simulink model "Robot_2R_Dynamics_and_Control"  (R2025a)
settings: Solver=ode4  StartTime=0.0  StopTime=stpt  FixedStep=0.001  MaxStep=0.001  MinStep=1e-6  RelTol=1e-3
undefined symbols (not defined in the file): acceleration, c, position, velocity, x, xx
libraries: slpidlib x2
settings Model: SimulationMode=accelerator  Creator=davi_  LastModifiedBy=GrupoGarra
settings DebuggingCC: UnconnectedInputMsg=warning  UnconnectedOutputMsg=warning  UnconnectedLineMsg=warning
settings ModelReferenceCC: EnableRefExpFcnMdlSchedulingChecks=on
settings RTWCC: GPUComputeCapability=3.5  DLArmComputeVersion=19.05

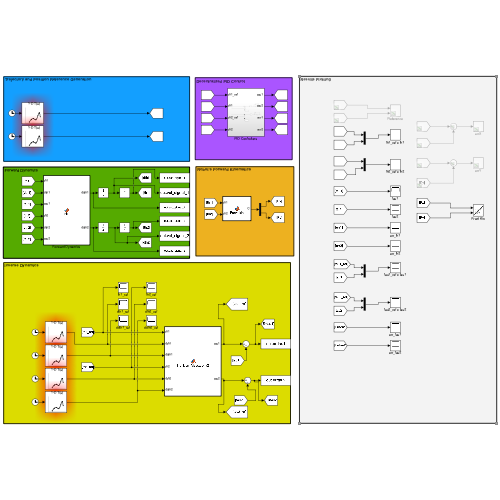
[thumbnail: Simulink's stored preview of the top-level diagram]
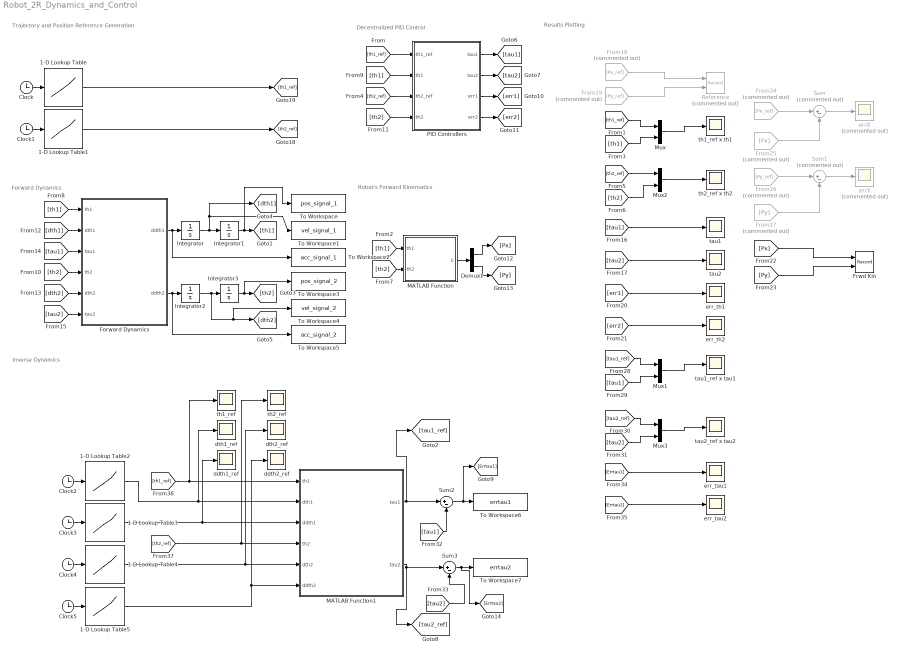
== system Robot_2R_Dynamics_and_Control ==
  note: Inverse Dynamics
  note: Results Plotting
  note: Forward Dynamics
  note: Robot's Forward Kinematics
  note: Trajectory and Position Reference Generation
  note: Decentralized PID Control
  1-D Lookup Table : Lookup_n-D  NumberOfTableDimensions=1  BreakpointsForDimension1=xx  Table=position(1,:)  InterpMethod=Cubic spline  ExtrapMethod=Clip  InternalRulePriority=Speed  RndMeth=Simplest
  1-D Lookup Table1 : Lookup_n-D  NumberOfTableDimensions=1  BreakpointsForDimension1=xx  Table=position(2,:)  InterpMethod=Cubic spline  ExtrapMethod=Clip  InternalRulePriority=Speed  RndMeth=Simplest
  1-D Lookup Table2 : Lookup_n-D  NumberOfTableDimensions=1  BreakpointsForDimension1=xx  Table=velocity(1,:)  InterpMethod=Cubic spline  ExtrapMethod=Clip  InternalRulePriority=Speed  RndMeth=Simplest
  1-D Lookup Table3 : Lookup_n-D  NumberOfTableDimensions=1  BreakpointsForDimension1=xx  Table=acceleration(1,:)  InterpMethod=Cubic spline  ExtrapMethod=Clip  InternalRulePriority=Speed  RndMeth=Simplest
  1-D Lookup Table4 : Lookup_n-D  NumberOfTableDimensions=1  BreakpointsForDimension1=xx  Table=velocity(2,:)  InterpMethod=Cubic spline  ExtrapMethod=Clip  InternalRulePriority=Speed  RndMeth=Simplest
  1-D Lookup Table5 : Lookup_n-D  NumberOfTableDimensions=1  BreakpointsForDimension1=xx  Table=acceleration(2,:)  InterpMethod=Cubic spline  ExtrapMethod=Clip  InternalRulePriority=Speed  RndMeth=Simplest
  Clock{,1..5} (6 alike) : Clock
  Demux1 : Demux  Outputs=2
  Forward Dynamics : MATLAB Function  TreatAsAtomicUnit=on
  From18 : From  Commented=on  GotoTag=Px_ref
  From19 : From  Commented=on  GotoTag=Py_ref
  From24 : From  Commented=on  GotoTag=Px_ref
  From25 : From  Commented=on  GotoTag=Px
  From26 : From  Commented=on  GotoTag=Py_ref
  From27 : From  Commented=on  GotoTag=Py
  Frwd Kin : Record  NumPorts=2.0  FileSettingsInternal="{\"entries\":[{\"content\":{\"excelSettings\":{\"content\":{},\"type\":\"Streamout.ExcelSettings\"},\"parquetSettings\":{\"content\":{},\"type\":\"Streamout.ParquetSettings\"}},\"type\":\"Streamout.FileSettingStorage\",\"uuid\":\"\"}],\"packageUris\":[\"http:\\/\\/schema.mathworks.com\\/mf0\\/streamout_blocks\\/R2020a\"],\"version\":\"1.0\"}"  FrameSettings=[0, 0]  Layout=[1 1]  SignalsInternal="{\"entries\":[{\"content\":{\"signals\":[{\"content\":{\"blockPath\":[],\"dimensions\":[1],\"domain\":\"\",\"lineColor\":\"#a2142f\",\"plots\":[ 1 ],\"port\":1,\"signalID\":1,\"signalName\":\"From22\"},\"type\":\"RecordBlkView.Signal\",\"uuid\":\"\"},{\"content\":{\"blockPath\":[],\"dimensions\":[1],\"domain\":\"\",\"lineColor\":\"#139fff\",\"plots\":[ 1 ],\"port\":2,\"signalID\":2,\"signalName\":\"From23\"},\"type\":\"RecordBlkView.Signal\",\"uuid\":\"\"}]},\"type\":\"RecordBlkView.InputSignals\",\"uuid\":\"\"}],\"packageUris\":[\"http:\\/\\/schema.mathworks.com\\/mf0\\/streamout_blocks\\/R2020a\"],\"version\":\"1.0\"}"  VisualizationBindings="{\"xyplotplugin\":{\"info\":[{\"series\":[{\"bindingParametersList\":[{\"parameter\":\"X-Axis\",\"signalID\":1,\"signalName\":\"From22\"},{\"parameter\":\"Y-Axis\",\"signalID\":2,\"signalName\":\"From23\"}],\"seriesID\":0}],\"subplotID\":1}]}}"  CompatibilityTag=XY  st=-1
  Integrator{,1..3} (4 alike) : Integrator
  MATLAB Function : MATLAB Function  TreatAsAtomicUnit=on
  MATLAB Function1 : MATLAB Function  TreatAsAtomicUnit=on
  Mux{,1..3} (4 alike) : Mux  Inputs=2
  PID Controllers : Subsystem
  Reference : Record  Commented=on  NumPorts=2.0  FileSettingsInternal="{\"entries\":[{\"content\":{\"excelSettings\":{\"content\":{},\"type\":\"Streamout.ExcelSettings\"},\"parquetSettings\":{\"content\":{},\"type\":\"Streamout.ParquetSettings\"}},\"type\":\"Streamout.FileSettingStorage\",\"uuid\":\"\"}],\"packageUris\":[\"http:\\/\\/schema.mathworks.com\\/mf0\\/streamout_blocks\\/R2020a\"],\"version\":\"1.0\"}"  FrameSettings=[0, 0]  Layout=[1 1]  SignalsInternal="{\"entries\":[{\"content\":{\"signals\":[{\"content\":{\"blockPath\":[],\"dimensions\":[1],\"domain\":\"\",\"lineColor\":\"#a2142f\",\"plots\":[ 1 ],\"port\":1,\"signalID\":1,\"signalName\":\"XY Graph:1\"},\"type\":\"RecordBlkView.Signal\",\"uuid\":\"\"},{\"content\":{\"blockPath\":[],\"dimensions\":[1],\"domain\":\"\",\"lineColor\":\"#139fff\",\"plots\":[ 1 ],\"port\":2,\"signalID\":2,\"signalName\":\"XY Graph:2\"},\"type\":\"RecordBlkView.Signal\",\"uuid\":\"\"}]},\"type\":\"RecordBlkView.InputSignals\",\"uuid\":\"\"}],\"packageUris\":[\"http:\\/\\/schema.mathworks.com\\/mf0\\/streamout_blocks\\/R2020a\"],\"version\":\"1.0\"}"  VisualizationBindings="{\"xyplotplugin\":{\"info\":[{\"series\":[{\"bindingParametersList\":[{\"parameter\":\"X-Axis\",\"signalID\":1,\"signalName\":\"XY Graph:1\"},{\"parameter\":\"Y-Axis\",\"signalID\":2,\"signalName\":\"XY Graph:2\"}],\"seriesID\":0}],\"subplotID\":1}]}}"  CompatibilityTag=XY  st=-1
  Sum : Sum  Commented=on  Inputs=|+-
  Sum1 : Sum  Commented=on  Inputs=|+-
  Sum2 : Sum  Inputs=|+-
  Sum3 : Sum  Inputs=|+-
  To Workspace : ToWorkspace  VariableName=pos_signal_1  SampleTime=-1
  To Workspace1 : ToWorkspace  VariableName=vel_signal_1  SampleTime=-1
  To Workspace2 : ToWorkspace  VariableName=acc_signal_1  SampleTime=-1
  To Workspace3 : ToWorkspace  VariableName=pos_signal_2  SampleTime=-1
  To Workspace4 : ToWorkspace  VariableName=vel_signal_2  SampleTime=-1
  To Workspace5 : ToWorkspace  VariableName=acc_signal_2  SampleTime=-1
  To Workspace6 : ToWorkspace  VariableName=errtau1  SampleTime=-1
  To Workspace7 : ToWorkspace  VariableName=errtau2  SampleTime=-1
  ddth1_ref : Scope
      settings: ActiveDisplayYMinimum=-1.7046  ActiveDisplayYMaximum=10.72886  DataLoggingVariableName=ScopeData2
  ddth2_ref : Scope
      settings: ActiveDisplayYMinimum=-29.79825  ActiveDisplayYMaximum=6.00469  DataLoggingVariableName=ScopeData3
  dth1_ref : Scope
      settings: ActiveDisplayYMinimum=-0.76549  ActiveDisplayYMaximum=1.78872
  dth2_ref : Scope
      settings: ActiveDisplayYMinimum=-0.46079  ActiveDisplayYMaximum=1.47482  DataLoggingVariableName=ScopeData5
  errX : Scope  Commented=on
      settings: ActiveDisplayYMinimum=-0.05671  ActiveDisplayYMaximum=0.09104  DataLoggingVariableName=ScopeData5
  errY : Scope  Commented=on
      settings: ActiveDisplayYMinimum=-0.05671  ActiveDisplayYMaximum=0.09104  DataLoggingVariableName=ScopeData6
  err_tau1 : Scope
      settings: ActiveDisplayYMinimum=-0.10365664078186178  ActiveDisplayYMaximum=0.12157927180851377
  err_tau2 : Scope
      settings: ActiveDisplayYMinimum=-0.11596  ActiveDisplayYMaximum=0.12339  DataLoggingVariableName=ScopeData2
  err_th1 : Scope
      settings: ActiveDisplayYMinimum=-0.0011718016150849826  ActiveDisplayYMaximum=0.000974877138754193  DataLoggingVariableName=ScopeData2
  err_th2 : Scope
      settings: ActiveDisplayYMinimum=-0.46542  ActiveDisplayYMaximum=0.0529
  tau1 : Scope
      settings: ActiveDisplayYMinimum=-21.92284  ActiveDisplayYMaximum=23.22624  DataLoggingVariableName=ScopeData3
  tau1_ref x tau1 : Scope
      settings: ActiveDisplayYMinimum=-22.72078  ActiveDisplayYMaximum=23.87515
  tau2 : Scope
      settings: ActiveDisplayYMinimum=-3.67368  ActiveDisplayYMaximum=4.67521  DataLoggingVariableName=ScopeData4
  tau2_ref x tau2 : Scope
      settings: ActiveDisplayYMinimum=-16.2578  ActiveDisplayYMaximum=18.66466  DataLoggingVariableName=ScopeData2
  th1_ref : Scope
      settings: ActiveDisplayYMinimum=-0.4737  ActiveDisplayYMaximum=1.16382  DataLoggingVariableName=ScopeData3
  th1_ref x th1 : Scope
      settings: ActiveDisplayYMinimum=-0.47526  ActiveDisplayYMaximum=1.16405
  th2_ref : Scope
      settings: ActiveDisplayYMinimum=-0.98175  ActiveDisplayYMaximum=0.98175  DataLoggingVariableName=ScopeData4
  th2_ref x th2 : Scope
      settings: ActiveDisplayYMinimum=-0.14358  ActiveDisplayYMaximum=1.2922  DataLoggingVariableName=ScopeData7
  wires:
  Forward Dynamics/1(ddth1) -> To Workspace2/1, Integrator/1
  Integrator/1 -> To Workspace1/1, [dth1], Integrator1/1
  Integrator1/1 -> To Workspace/1, [th1]
  Forward Dynamics/2(ddth2) -> To Workspace5/1, Integrator2/1
  Integrator2/1 -> To Workspace4/1, [dth2], Integrator3/1
  Integrator3/1 -> To Workspace3/1, [th2]
  Mux/1 -> th1_ref x th1/1
  Sum/1 -> errX/1
  Sum1/1 -> errY/1
  [th1_ref] -> Mux/1
  [th1] -> MATLAB Function/1(th1)
  [th1] -> Mux/2
  [th2] -> Mux2/2
  [th2_ref] -> Mux2/1
  Mux2/1 -> th2_ref x th2/1
  [th2] -> MATLAB Function/2(th2)
  [th1] -> Forward Dynamics/1(th1)
  [th2] -> Forward Dynamics/4(th2)
  [dth1] -> Forward Dynamics/2(dth1)
  [dth2] -> Forward Dynamics/5(dth2)
  [tau1] -> Forward Dynamics/3(tau1)
  [tau2] -> Forward Dynamics/6(tau2)
  [tau1] -> tau1/1
  [tau2] -> tau2/1
  From18/1 -> Reference/1
  From19/1 -> Reference/2
  [err1] -> err_th1/1
  [err2] -> err_th2/1
  MATLAB Function/1(C) -> Demux1/1
  Demux1/2 -> [Py]
  Demux1/1 -> [Px]
  [Px] -> Frwd Kin/1
  [Py] -> Frwd Kin/2
  From24/1 -> Sum/1
  From25/1 -> Sum/2
  From26/1 -> Sum1/1
  From27/1 -> Sum1/2
  PID Controllers/4(err2) -> [err2]
  [th2] -> PID Controllers/4(th2)
  PID Controllers/1(tau1) -> [tau1]
  PID Controllers/2(tau2) -> [tau2]
  [th1_ref] -> PID Controllers/1(th1_ref)
  PID Controllers/3(err1) -> [err1]
  [th2_ref] -> PID Controllers/3(th2_ref)
  [th1] -> PID Controllers/2(th1)
  1-D Lookup Table/1 -> [th1_ref]
  1-D Lookup Table1/1 -> [th2_ref]
  1-D Lookup Table2/1 -> MATLAB Function1/2(dth1), dth1_ref/1
  MATLAB Function1/2(tau2) -> Sum3/1, [tau2_ref]
  1-D Lookup Table4/1 -> MATLAB Function1/5(dth2), dth2_ref/1
  [th2_ref] -> th2_ref/1, MATLAB Function1/4(th2)
  1-D Lookup Table5/1 -> MATLAB Function1/6(ddth2), ddth2_ref/1
  1-D Lookup Table3/1 -> MATLAB Function1/3(ddth1), ddth1_ref/1
  MATLAB Function1/1(tau1) -> Sum2/1, [tau1_ref]
  [tau1_ref] -> Mux1/1
  [tau1] -> Mux1/2
  Mux1/1 -> tau1_ref x tau1/1
  Mux3/1 -> tau2_ref x tau2/1
  [tau2] -> Mux3/2
  [tau2_ref] -> Mux3/1
  [tau1] -> Sum2/2
  [tau2] -> Sum3/2
  Sum2/1 -> To Workspace6/1, [Errtau1]
  Sum3/1 -> To Workspace7/1, [Errtau2]
  [Errtau2] -> err_tau2/1
  [Errtau1] -> err_tau1/1
  Clock/1 -> 1-D Lookup Table/1
  Clock1/1 -> 1-D Lookup Table1/1
  [th1_ref] -> th1_ref/1, MATLAB Function1/1(th1)
  Clock2/1 -> 1-D Lookup Table2/1
  Clock3/1 -> 1-D Lookup Table3/1
  Clock4/1 -> 1-D Lookup Table4/1
  Clock5/1 -> 1-D Lookup Table5/1

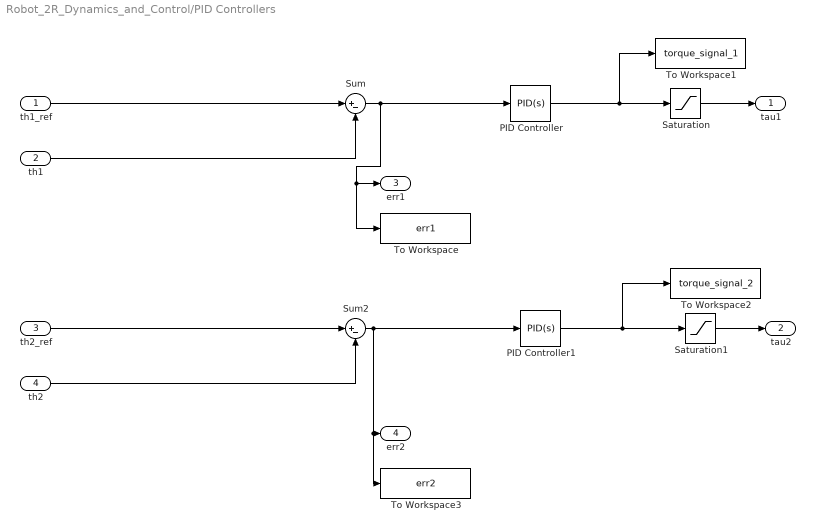
== system Robot_2R_Dynamics_and_Control/PID Controllers ==
  th1_ref : Inport
  th1 : Inport  Port=2
  th2_ref : Inport  Port=3
  th2 : Inport  Port=4
  PID Controller : slpidlib/PID Controller  Controller=PID  Form=Parallel  TimeDomain=Continuous-time  UseExternalTs=off  SampleTime=-1  IntegratorMethod=Forward Euler  FilterMethod=Forward Euler  ControllerParametersSource=internal  P=x(1)  I=x(3)  UseKiTs=off  D=x(2)  UseExternalDerivativeSource=off  N=c  UseFilter=on  TunerSelectOption=Transfer Function Based (PID Tuner App)  InitialConditionSource=internal  InitialConditionForIntegrator=0  InitialConditionForFilter=0  DifferentiatorICPrevScaledInput=0  ExternalReset=none  TrackingMode=off  Kt=1  LimitOutput=off  SatLimitsSource=internal  UpperSaturationLimit=inf  LowerSaturationLimit=-inf  LinearizeAsGain=on  AntiWindupMode=none  Kb=1  LimitIntegrator=off  UpperIntegratorSaturationLimit=inf  LowerIntegratorSaturationLimit=-inf  POutMin=[]  POutMax=[]  IOutMin=[]  IOutMax=[]  DOutMin=[]  DOutMax=[]  NOutMin=[]  NOutMax=[]  SumOutMin=[]  SumOutMax=[]  SaturationOutMin=[]  SaturationOutMax=[]  PParamMin=[]  PParamMax=[]  IParamMin=[]  IParamMax=[]  DParamMin=[]  DParamMax=[]  NParamMin=[]  NParamMax=[]  KbParamMin=[]  KbParamMax=[]  KtParamMin=[]  KtParamMax=[]  KbOutMin=[]  KbOutMax=[]  KtOutMin=[]  KtOutMax=[]  IntegratorOutMin=[]  IntegratorOutMax=[]  FilterOutMin=[]  FilterOutMax=[]  SumI1OutMin=[]  SumI1OutMax=[]  SumI2OutMin=[]  SumI2OutMax=[]  SumI3OutMin=[]  SumI3OutMax=[]  SumI4OutMin=[]  SumI4OutMax=[]  SumDOutMin=[]  SumDOutMax=[]  DifferentiatorOutMin=[]  DifferentiatorOutMax=[]  FilterDiffOutCoefMin=[]  FilterDiffOutCoefMax=[]  ReciprocalOutMin=[]  ReciprocalOutMax=[]  SumDenOutMin=[]  SumDenOutMax=[]  SumNumOutMin=[]  SumNumOutMax=[]  DivideOutMin=[]  DivideOutMax=[]  UdiffTsProdOutMin=[]  UdiffTsProdOutMax=[]  NTsProdOutMin=[]  NTsProdOutMax=[]  UintegralTsProdOutMin=[]  UintegralTsProdOutMax=[]  UngainTsProdOutMin=[]  UngainTsProdOutMax=[]  ClampingZeroOutDataTypeStr=Inherit: Inherit via back propagation  ClampingZeroOutMin=[]  ClampingZeroOutMax=[]  FilterDenConstantOutDataTypeStr=Inherit: Inherit via back propagation  FilterDenConstantOutMin=[]  FilterDenConstantOutMax=[]  PCopyOutDataTypeStr=Inherit: Inherit via back propagation  PCopyOutMin=[]  PCopyOutMax=[]  NCopyOutDataTypeStr=Inherit: Inherit via back propagation  NCopyOutMin=[]  NCopyOutMax=[]  IntegratorContinuousStateAttributes=''  IntegratorStateMustResolveToSignalObject=off  IntegratorRTWStateStorageClass=Auto  FilterContinuousStateAttributes=''  FilterStateMustResolveToSignalObject=off  FilterRTWStateStorageClass=Auto  ParallelPVariant=InternalParameters  IdealPVariant=Disabled  IVariant=InternalParameters  DVariant=InternalParameters  IntegratorVariant=Continuous  SatVariant=Disabled  AWVariant=Passthrough  PCopyVariant=Disabled  TRVariant=Disabled  FdbkBlocksVariant=Forward  IdealPFdbkVariant=Disabled  SatFdbkVariant=Disabled  DerivativeFilterVariant=ContFilter  NVariant=InternalParameters  NCopyVariant=Disabled  FilterICVariant=InternalICsFilter  IntegratorICVariant=InternalICs  ExternalResetVariant=Disabled  TRSumVariant=Passthrough  SumFdbkVariant=Disabled  SumVariant=Sum_PID  TsampFilterVariant=InternalTs  TsampNgainVariant=Passthrough  TsampIntegralVariant=Disabled_SignalSpec  ExternalSaturationOutDataTypeStr=Inherit: Same as second input  DerivativeSourceVariant=ErrorSignal  PreIntVariant=InternalPreInt
  PID Controller1 : slpidlib/PID Controller  Controller=PID  Form=Parallel  TimeDomain=Continuous-time  UseExternalTs=off  SampleTime=-1  IntegratorMethod=Forward Euler  FilterMethod=Forward Euler  ControllerParametersSource=internal  P=x(4)  I=x(6)  UseKiTs=off  D=x(5)  UseExternalDerivativeSource=off  N=c  UseFilter=on  TunerSelectOption=Transfer Function Based (PID Tuner App)  InitialConditionSource=internal  InitialConditionForIntegrator=0  InitialConditionForFilter=0  DifferentiatorICPrevScaledInput=0  ExternalReset=none  TrackingMode=off  Kt=1  LimitOutput=off  SatLimitsSource=internal  UpperSaturationLimit=inf  LowerSaturationLimit=-inf  LinearizeAsGain=on  AntiWindupMode=none  Kb=1  LimitIntegrator=off  UpperIntegratorSaturationLimit=inf  LowerIntegratorSaturationLimit=-inf  POutMin=[]  POutMax=[]  IOutMin=[]  IOutMax=[]  DOutMin=[]  DOutMax=[]  NOutMin=[]  NOutMax=[]  SumOutMin=[]  SumOutMax=[]  SaturationOutMin=[]  SaturationOutMax=[]  PParamMin=[]  PParamMax=[]  IParamMin=[]  IParamMax=[]  DParamMin=[]  DParamMax=[]  NParamMin=[]  NParamMax=[]  KbParamMin=[]  KbParamMax=[]  KtParamMin=[]  KtParamMax=[]  KbOutMin=[]  KbOutMax=[]  KtOutMin=[]  KtOutMax=[]  IntegratorOutMin=[]  IntegratorOutMax=[]  FilterOutMin=[]  FilterOutMax=[]  SumI1OutMin=[]  SumI1OutMax=[]  SumI2OutMin=[]  SumI2OutMax=[]  SumI3OutMin=[]  SumI3OutMax=[]  SumI4OutMin=[]  SumI4OutMax=[]  SumDOutMin=[]  SumDOutMax=[]  DifferentiatorOutMin=[]  DifferentiatorOutMax=[]  FilterDiffOutCoefMin=[]  FilterDiffOutCoefMax=[]  ReciprocalOutMin=[]  ReciprocalOutMax=[]  SumDenOutMin=[]  SumDenOutMax=[]  SumNumOutMin=[]  SumNumOutMax=[]  DivideOutMin=[]  DivideOutMax=[]  UdiffTsProdOutMin=[]  UdiffTsProdOutMax=[]  NTsProdOutMin=[]  NTsProdOutMax=[]  UintegralTsProdOutMin=[]  UintegralTsProdOutMax=[]  UngainTsProdOutMin=[]  UngainTsProdOutMax=[]  ClampingZeroOutDataTypeStr=Inherit: Inherit via back propagation  ClampingZeroOutMin=[]  ClampingZeroOutMax=[]  FilterDenConstantOutDataTypeStr=Inherit: Inherit via back propagation  FilterDenConstantOutMin=[]  FilterDenConstantOutMax=[]  PCopyOutDataTypeStr=Inherit: Inherit via back propagation  PCopyOutMin=[]  PCopyOutMax=[]  NCopyOutDataTypeStr=Inherit: Inherit via back propagation  NCopyOutMin=[]  NCopyOutMax=[]  IntegratorContinuousStateAttributes=''  IntegratorStateMustResolveToSignalObject=off  IntegratorRTWStateStorageClass=Auto  FilterContinuousStateAttributes=''  FilterStateMustResolveToSignalObject=off  FilterRTWStateStorageClass=Auto  ParallelPVariant=InternalParameters  IdealPVariant=Disabled  IVariant=InternalParameters  DVariant=InternalParameters  IntegratorVariant=Continuous  SatVariant=Disabled  AWVariant=Passthrough  PCopyVariant=Disabled  TRVariant=Disabled  FdbkBlocksVariant=Forward  IdealPFdbkVariant=Disabled  SatFdbkVariant=Disabled  DerivativeFilterVariant=ContFilter  NVariant=InternalParameters  NCopyVariant=Disabled  FilterICVariant=InternalICsFilter  IntegratorICVariant=InternalICs  ExternalResetVariant=Disabled  TRSumVariant=Passthrough  SumFdbkVariant=Disabled  SumVariant=Sum_PID  TsampFilterVariant=InternalTs  TsampNgainVariant=Passthrough  TsampIntegralVariant=Disabled_SignalSpec  ExternalSaturationOutDataTypeStr=Inherit: Same as second input  DerivativeSourceVariant=ErrorSignal  PreIntVariant=InternalPreInt
  Saturation : Saturate  UpperLimit=25  LowerLimit=-25
  Saturation1 : Saturate  UpperLimit=9  LowerLimit=-9
  Sum : Sum  Inputs=|+-
  Sum2 : Sum  Inputs=|+-
  To Workspace : ToWorkspace  VariableName=err1  SampleTime=-1
  To Workspace1 : ToWorkspace  VariableName=torque_signal_1  SampleTime=-1
  To Workspace2 : ToWorkspace  VariableName=torque_signal_2  SampleTime=-1
  To Workspace3 : ToWorkspace  VariableName=err2  SampleTime=-1
  tau1 : Outport
  tau2 : Outport  Port=2
  err1 : Outport  Port=3
  err2 : Outport  Port=4
  wires:
  Sum/1 -> PID Controller/1, To Workspace/1, err1/1
  th2_ref/1 -> Sum2/1
  th2/1 -> Sum2/2
  th1_ref/1 -> Sum/1
  th1/1 -> Sum/2
  PID Controller/1 -> To Workspace1/1, Saturation/1
  Saturation/1 -> tau1/1
  Saturation1/1 -> tau2/1
  Sum2/1 -> PID Controller1/1, To Workspace3/1, err2/1
  PID Controller1/1 -> To Workspace2/1, Saturation1/1

== matlab function Robot_2R_Dynamics_and_Control/MATLAB Function1 ==
  data: th1 input; tau1 output; dth1 input; ddth1 input; th2 input; dth2 input; ddth2 input; tau2 output
function [tau1, tau2] = Inv_Dyn_Massaro_v2(th1, dth1, ddth1, th2, dth2, ddth2)
    
    
    L1 = 0.4; % length of link 1 (m)         
    L2 = 0.25; % length of link 2 (m)

    m1 = 29.58; % mass of link 1 (kg)
    m2 = 15; % mass of link 2 (kg)
    Ml = 6; % mass of the payload (kg)
    
    I1 = 0.417;
    I2 = 0.206;
    
    b1 = L1/2;
    b2 = L2/2;

    alpha = I1 + I2 + m1*b1^2 + m2*(L1^2 + b2^2) + Ml*(L1^2+L2^2); % constant base inertia
    gamma = I2 + m2*b2^2 + Ml*L2^2; % constant end effector inertia
    beta = m2*L1*b2 + Ml*L1*L2; % cooupling coefficient
    
    M = [alpha + 2*beta*cos(th2) gamma + beta*cos(th2);
         gamma + beta*cos(th2)         gamma          ]; % mass matrix

    C = [-beta*sin(th2)*dth2 -beta*sin(th2)*(dth1+dth2);
          beta*sin(th2)*dth1            0             ]; % coriolis and centrifugal force matrix

%     G = [gc*(((1/2)*m1 + m2)*L1*cos(th1) + (1/2)*m2*L2*cos(th1+th2));
%          (1/2)*m2*gc*L2*cos(th1+th2)]; % gravitational force matrix

%     F = [0;0]; % friction force matrix
    dTH = [dth1;dth2];
    ddTH = [ddth1;ddth2];

    
  T = M*ddTH + C*dTH;
  tau1 = T(1);
  tau2 = T(2);

== matlab function Robot_2R_Dynamics_and_Control/MATLAB Function ==
  data: th1 input; C output; th2 input
function C  = Forw_kin(th1,th2)

L1 = 0.4; % length of link 1 (m)         
L2 = 0.25; % length of link 2 (m)

C = [L1*cos(th1)+L2*cos(th1+th2);L1*sin(th1)+...
     L2*sin(th1+th2)]; % coordinates of point C written in 
                       % the inertial reference frame(m)
end

== matlab function Robot_2R_Dynamics_and_Control/Forward Dynamics ==
  data: th1 input; ddth1 output; dth1 input; tau1 input; th2 input; dth2 input; tau2 input; ddth2 output
function [ddth1, ddth2] = NE(th1, dth1, tau1, th2, dth2, tau2)
    L1 = 0.4; % length of link 1 (m)         
    L2 = 0.25; % length of link 2 (m)

    m1 = 29.58; % mass of link 1 (kg)
    m2 = 15; % mass of link 2 (kg)
    Ml = 6; % mass of the payload (kg)
    
    I1 = 0.417;
    I2 = 0.206;
    
    b1 = L1/2;
    b2 = L2/2;

    alpha = I1 + I2 + m1*b1^2 + m2*(L1^2 + b2^2) + Ml*(L1^2+L2^2); % constant base inertia phi
    gamma = I2 + m2*b2^2 + Ml*L2^2; % constant end effector inertia rho
    beta = m2*L1*b2 + Ml*L1*L2; % cooupling coefficient psi
    
    M = [alpha + 2*beta*cos(th2) gamma + beta*cos(th2);
         gamma + beta*cos(th2)         gamma          ]; % mass matrix

    C = [-beta*sin(th2)*dth2 -beta*sin(th2)*(dth1+dth2);
          beta*sin(th2)*dth1            0             ]; % coriolis and centrifugal force matrix
    T = [tau1;tau2];
    dTH = [dth1;dth2];

    ddTH = M\(T - (C*dTH));
    
    ddth1 = ddTH(1);
    ddth2 = ddTH(2);
